simulink model "voll_bridge_tobias"  (R2026b)
settings: Solver=VariableStepAuto
undefined symbols (not defined in the file): C_in_filter, Delta, L, L1, L2, L_in_filter, Lm, N, n, N_points, R1, R2, R_in_filter, RFe, RLrp, TA
libraries: simulink x6, SDE_Blockset x1
settings Model: Creator=trainer  LastModifiedBy=d.bagnara
settings OptimizationCC: ReuseModelBlockBuffer=off

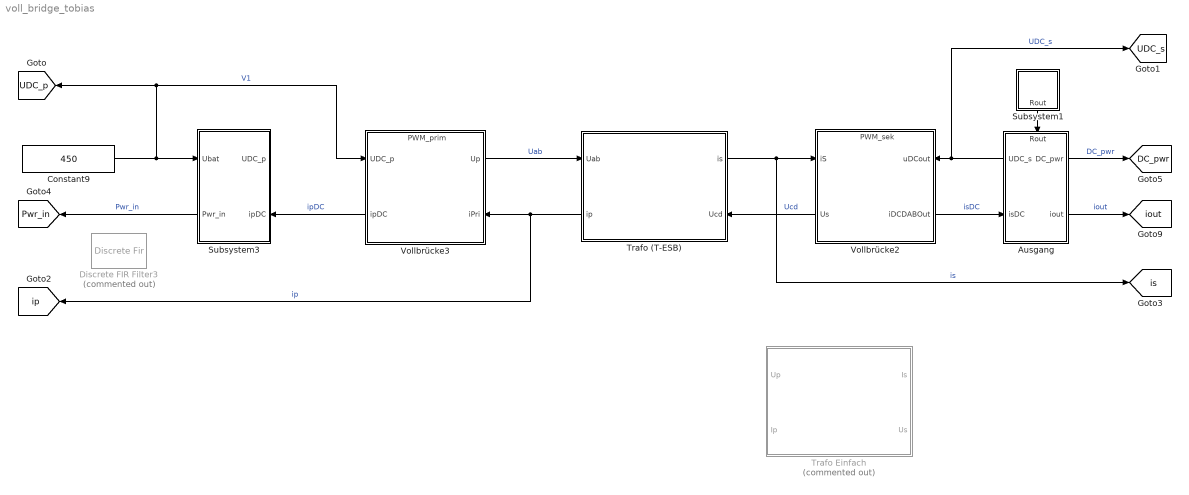
== system voll_bridge_tobias ==
  Ausgang : Subsystem
      settings: PortSchema="{\"entries\":[{\"content\":{\"sides\":[{\"content\":{\"connectorIds\":[\"Out3\",\"In1\"]},\"type\":\"ConnectorPlacement.EquallySpacedRectSide\",\"uuid\":\"3e2cff53-c875-49c6-8474-afa1ed1193a6\"},{\"content\":{\"connectorIds\":[\"Out1\",\"Out2\"],\"side\":\"RIGHT\"},\"type\":\"ConnectorPlacement.EquallySpacedRectSide\",\"uuid\":\"9e2ae12c-269a-4542-b310-d161ff5322e5\"},{\"content\":{\"connectorIds\":[\"In2\"],\"side\":\"TOP\"},\"type\":\"ConnectorPlacement.EquallySpacedRectSide\",\"uuid\":\"7466d0b4-47a5-439f-b3f3-5fed0d3de2ac\"}]},\"type\":\"ConnectorPlacement.EquallySpacedConnector\",\"uuid\":\"f94e0f93-850d-4090-9895-e2c6fde01ad6\"}],\"packageUris\":[\"http://schema.mathworks.com/mf0/Connector/R2020b\"],\"version\":\"1.0\"}"
  Constant9 : Constant  Value=450  OutDataTypeStr=S_F32
  Discrete FIR Filter3 : DiscreteFir  Commented=on  Coefficients=ones(1,N_points)/N_points  OutDataTypeStr=Inherit: Same as accumulator
  Subsystem1 : Subsystem
  Subsystem3 : Subsystem
      settings: PortSchema="{\"entries\":[{\"content\":{\"sides\":[{\"content\":{\"connectorIds\":[\"In1\",\"Out2\"]},\"type\":\"ConnectorPlacement.EquallySpacedRectSide\",\"uuid\":\"80c5ed0c-5841-4938-b898-84137f6d9c34\"},{\"content\":{\"connectorIds\":[\"Out1\",\"In2\"],\"side\":\"RIGHT\"},\"type\":\"ConnectorPlacement.EquallySpacedRectSide\",\"uuid\":\"8c17f11a-4998-4b66-b746-a293eee14202\"},{\"content\":{\"connectorIds\":[],\"side\":\"TOP\"},\"type\":\"ConnectorPlacement.EquallySpacedRectSide\",\"uuid\":\"e60db4c2-c92c-402f-8091-b49c7a789db5\"}]},\"type\":\"ConnectorPlacement.EquallySpacedConnector\",\"uuid\":\"558de1e2-c2ec-4343-96f3-e5efd467d9a7\"}],\"packageUris\":[\"http://schema.mathworks.com/mf0/Connector/R2020b\"],\"version\":\"1.0\"}"
  Trafo (T-ESB) : Subsystem
      settings: PortSchema="{\"entries\":[{\"content\":{\"sides\":[{\"content\":{\"connectorIds\":[\"In1\",\"Out2\"]},\"type\":\"ConnectorPlacement.EquallySpacedRectSide\",\"uuid\":\"6e81ceeb-0363-463f-984b-d2d8288a5ec4\"},{\"content\":{\"connectorIds\":[\"Out1\",\"In2\"],\"side\":\"RIGHT\"},\"type\":\"ConnectorPlacement.EquallySpacedRectSide\",\"uuid\":\"b30afd59-af09-43dc-9a37-2f5643c5d178\"},{\"content\":{\"connectorIds\":[],\"side\":\"TOP\"},\"type\":\"ConnectorPlacement.EquallySpacedRectSide\",\"uuid\":\"a71b4fb2-5a5a-43bb-9a64-a7dea3e55af5\"}]},\"type\":\"ConnectorPlacement.EquallySpacedConnector\",\"uuid\":\"85fc6124-daf2-4d92-a632-153b83626f2a\"}],\"packageUris\":[\"http://schema.mathworks.com/mf0/Connector/R2020b\"],\"version\":\"1.0\"}"
  Trafo Einfach : Subsystem  Commented=on
      settings: PortSchema="{\"entries\":[{\"content\":{\"sides\":[{\"content\":{\"connectorIds\":[\"In1\",\"Out2\"]},\"type\":\"ConnectorPlacement.EquallySpacedRectSide\",\"uuid\":\"c971f182-6d77-4937-8b05-b79f55e4c806\"},{\"content\":{\"connectorIds\":[\"Out1\",\"In2\"],\"side\":\"RIGHT\"},\"type\":\"ConnectorPlacement.EquallySpacedRectSide\",\"uuid\":\"37e64967-fcec-4802-beb3-69154f28263c\"},{\"content\":{\"connectorIds\":[],\"side\":\"TOP\"},\"type\":\"ConnectorPlacement.EquallySpacedRectSide\",\"uuid\":\"e411a49c-daa7-47d0-8386-3b1061192469\"},{\"content\":{\"connectorIds\":[],\"side\":\"BOTTOM\"},\"type\":\"ConnectorPlacement.EquallySpacedRectSide\",\"uuid\":\"ba50093e-ff36-4075-81bf-05719850c996\"}]},\"type\":\"ConnectorPlacement.EquallySpacedConnector\",\"uuid\":\"82c6f70e-365e-41e7-aef8-e59438ced761\"}],\"packageUris\":[\"http://schema.mathworks.com/mf0/Connector/R2020b\"],\"version\":\"1.0\"}"
  Vollbrücke2 : Subsystem
      settings: PortSchema="{\"entries\":[{\"content\":{\"sides\":[{\"content\":{\"connectorIds\":[\"In1\",\"Out2\"]},\"type\":\"ConnectorPlacement.EquallySpacedRectSide\",\"uuid\":\"b2581c16-97fc-43c2-9374-a6229b1b4c11\"},{\"content\":{\"connectorIds\":[\"In3\",\"Out1\"],\"side\":\"RIGHT\"},\"type\":\"ConnectorPlacement.EquallySpacedRectSide\",\"uuid\":\"06f310f8-024e-445b-b4e4-58d56c4e10df\"},{\"content\":{\"connectorIds\":[\"In2\"],\"side\":\"TOP\"},\"type\":\"ConnectorPlacement.EquallySpacedRectSide\",\"uuid\":\"c56b8861-8968-41d2-9579-8e1534e46433\"}]},\"type\":\"ConnectorPlacement.EquallySpacedConnector\",\"uuid\":\"550ed9c8-70a1-48c7-a2e5-e55cd52d4178\"}],\"packageUris\":[\"http://schema.mathworks.com/mf0/Connector/R2020b\"],\"version\":\"1.0\"}"
  Vollbrücke3 : Subsystem
      settings: PortSchema="{\"entries\":[{\"content\":{\"sides\":[{\"content\":{\"connectorIds\":[\"In1\",\"Out2\"]},\"type\":\"ConnectorPlacement.EquallySpacedRectSide\",\"uuid\":\"b2581c16-97fc-43c2-9374-a6229b1b4c11\"},{\"content\":{\"connectorIds\":[\"Out1\",\"In3\"],\"side\":\"RIGHT\"},\"type\":\"ConnectorPlacement.EquallySpacedRectSide\",\"uuid\":\"06f310f8-024e-445b-b4e4-58d56c4e10df\"},{\"content\":{\"connectorIds\":[\"In2\"],\"side\":\"TOP\"},\"type\":\"ConnectorPlacement.EquallySpacedRectSide\",\"uuid\":\"c56b8861-8968-41d2-9579-8e1534e46433\"}]},\"type\":\"ConnectorPlacement.EquallySpacedConnector\",\"uuid\":\"550ed9c8-70a1-48c7-a2e5-e55cd52d4178\"}],\"packageUris\":[\"http://schema.mathworks.com/mf0/Connector/R2020b\"],\"version\":\"1.0\"}"
  tag scope: DC_pwr=global, Pwr_in=global, UDC_p=global, UDC_s=global, iout=global, ip=global, is=global
  wires:
  Trafo (T-ESB)/1(is) -> [is], Vollbrücke2/1(iS)  "is"
  Trafo (T-ESB)/2(ip) -> [ip], Vollbrücke3/3(iPri)  "ip"
  Subsystem1/1(Rout) -> Ausgang/2(Rout)
  Vollbrücke3/1(Up) -> Trafo (T-ESB)/1(Uab)  "Uab"
  Ausgang/2(iout) -> [iout]  "iout"
  Vollbrücke2/2(Us) -> Trafo (T-ESB)/2(Ucd)  "Ucd"
  Vollbrücke2/1(iDCDABOut) -> Ausgang/1(isDC)  "isDC"
  Constant9/1 -> [UDC_p], Vollbrücke3/1(UDC_p), Subsystem3/1(Ubat)  "V1"
  Vollbrücke3/2(ipDC) -> Subsystem3/2(ipDC)  "ipDC"
  Ausgang/1(DC_pwr) -> [DC_pwr]  "DC_pwr"
  Ausgang/3(UDC_s) -> [UDC_s], Vollbrücke2/3(uDCout)  "UDC_s"
  Subsystem3/2(Pwr_in) -> [Pwr_in]  "Pwr_in"

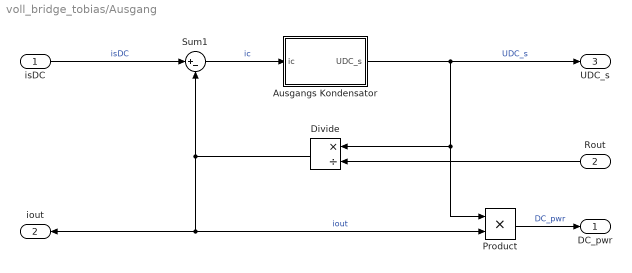
== system voll_bridge_tobias/Ausgang ==
  isDC : Inport
  Rout : Inport  Port=2
  Ausgangs Kondensator : Subsystem
  Divide : Product  Inputs=*/
  Product : Product
  Sum1 : Sum  Inputs=|+-
  DC_pwr : Outport
  iout : Outport  Port=2
  UDC_s : Outport  Port=3
  wires:
  Sum1/1 -> Ausgangs Kondensator/1(ic)  "ic"
  isDC/1 -> Sum1/1  "isDC"
  Divide/1 -> iout/1, Product/2, Sum1/2  "iout"
  Ausgangs Kondensator/1(UDC_s) -> UDC_s/1, Divide/1, Product/1  "UDC_s"
  Product/1 -> DC_pwr/1  "DC_pwr"
  Rout/1 -> Divide/2

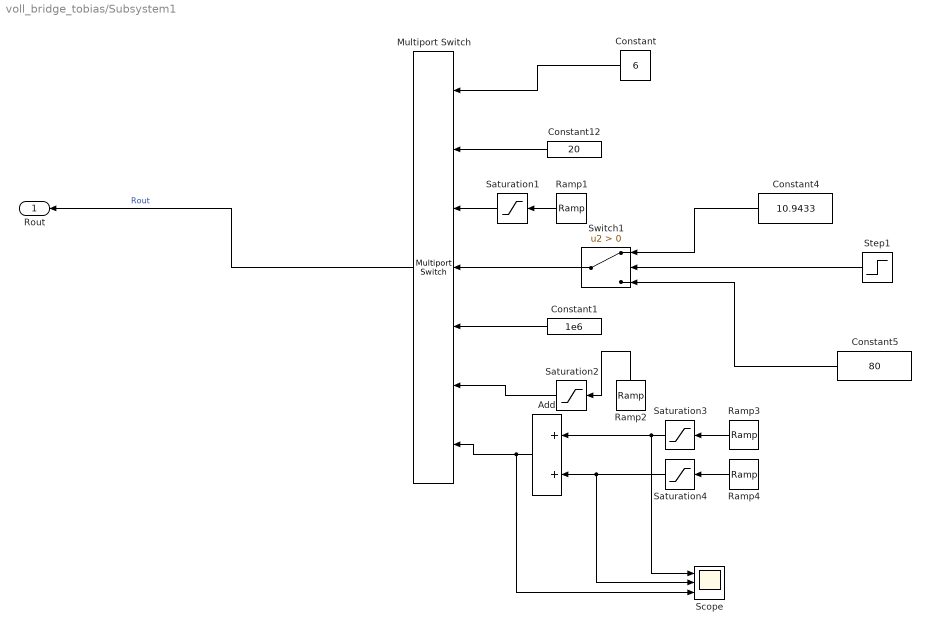
== system voll_bridge_tobias/Subsystem1 ==
  Add : Sum
  Constant : Constant  Value=6
  Constant1 : Constant  Value=1e6
  Constant12 : Constant  Value=20
  Constant4 : Constant  Value=10.9433
  Constant5 : Constant  Value=80
  Multiport Switch : SDE_Blockset/Signal Routing/Multiport Switch  DataPortOrder=One-based contiguous  Inputs=6  DataPortIndices={1,2,3}  DataPortForDefault=Last data port
      settings: SourceProductName=SDE_Blockset
  Ramp1 : simulink/Sources/Ramp  slope=-7450  start=0.005  InitialOutput=84.5
  Ramp2 : simulink/Sources/Ramp  slope=-1000  start=0.005  InitialOutput=20
  Ramp3 : simulink/Sources/Ramp  slope=-7450*2  start=0.005  InitialOutput=84.5
  Ramp4 : simulink/Sources/Ramp  slope=7450*2  start=0.02  InitialOutput=0
  Saturation1 : Saturate  UpperLimit=100  LowerLimit=10.9
  Saturation2 : Saturate  UpperLimit=100  LowerLimit=10.9
  Saturation3 : Saturate  UpperLimit=100  LowerLimit=10.9
  Saturation4 : Saturate  UpperLimit=84.5-10  LowerLimit=0
  Scope : Scope  NumInputPorts=3
      settings: ActiveDisplayYMinimum=1.7  ActiveDisplayYMaximum=93.7
  Step1 : Step  Time=0.005  SampleTime=0
  Switch1 : Switch  Criteria=u2 > Threshold  SaturateOnIntegerOverflow=off  InputSameDT=off
  Rout : Outport
  wires:
  Ramp1/1 -> Saturation1/1
  Constant4/1 -> Switch1/1
  Step1/1 -> Switch1/2
  Constant5/1 -> Switch1/3
  Constant12/1 -> Multiport Switch/2
  Saturation1/1 -> Multiport Switch/3
  Switch1/1 -> Multiport Switch/4
  Multiport Switch/1 -> Rout/1  "Rout"
  Constant/1 -> Multiport Switch/1
  Constant1/1 -> Multiport Switch/5
  Ramp2/1 -> Saturation2/1
  Saturation2/1 -> Multiport Switch/6
  Ramp3/1 -> Saturation3/1
  Add/1 -> Scope/3, Multiport Switch/7
  Saturation3/1 -> Scope/1, Add/1
  Saturation4/1 -> Scope/2, Add/2
  Ramp4/1 -> Saturation4/1

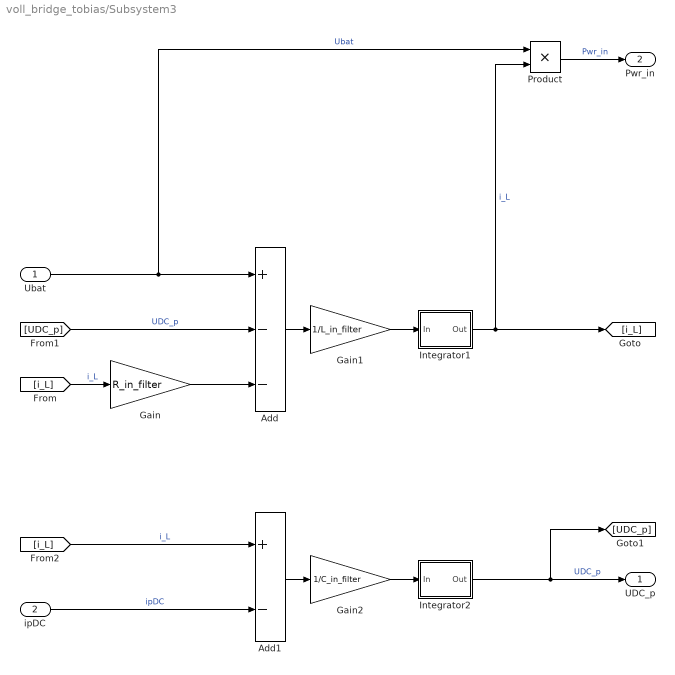
== system voll_bridge_tobias/Subsystem3 ==
  Ubat : Inport
  ipDC : Inport  Port=2
  Add : Sum  Inputs=+--
  Add1 : Sum  Inputs=+-
  Gain : Gain  Gain=R_in_filter
  Gain1 : Gain  Gain=1/L_in_filter
  Gain2 : Gain  Gain=1/C_in_filter
  Integrator1 : Subsystem
  Integrator2 : Subsystem
  Product : Product
  UDC_p : Outport
  Pwr_in : Outport  Port=2
  wires:
  Product/1 -> Pwr_in/1  "Pwr_in"
  ipDC/1 -> Add1/2  "ipDC"
  [i_L] -> Add1/1  "i_L"
  Gain2/1 -> Integrator2/1(In)
  Gain1/1 -> Integrator1/1(In)
  [UDC_p] -> Add/2  "UDC_p"
  [i_L] -> Gain/1  "i_L"
  Ubat/1 -> Add/1, Product/1  "Ubat"
  Add1/1 -> Gain2/1
  Integrator2/1(Out) -> UDC_p/1, [UDC_p]  "UDC_p"
  Integrator1/1(Out) -> [i_L], Product/2  "i_L"
  Add/1 -> Gain1/1
  Gain/1 -> Add/3

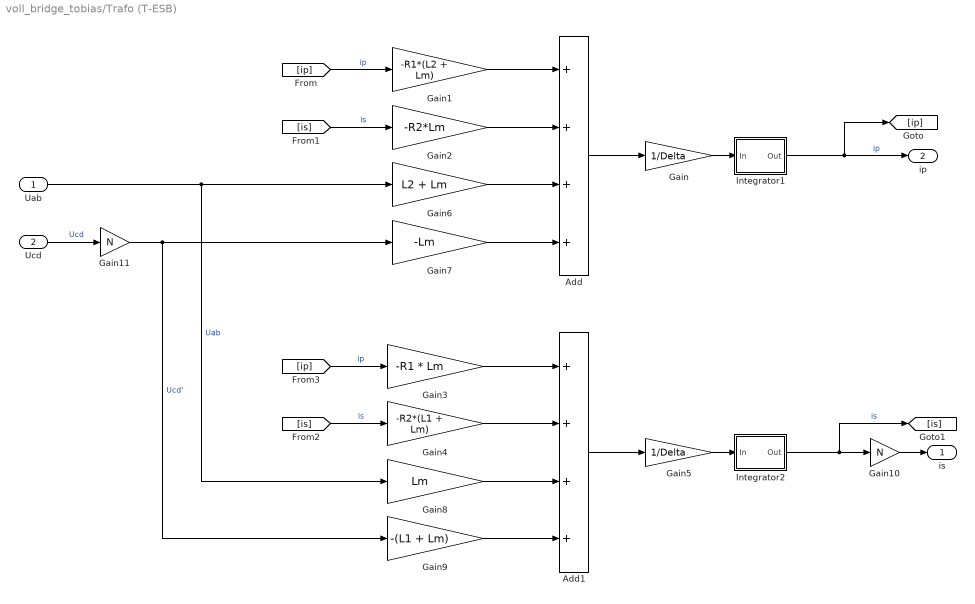
== system voll_bridge_tobias/Trafo (T-ESB) ==
  Uab : Inport
  Ucd : Inport  Port=2
  Add : Sum  Inputs=++++
  Add1 : Sum  Inputs=++++
  Gain : Gain  Gain=1/Delta
  Gain1 : Gain  Gain=-R1*(L2 + Lm)
  Gain10 : Gain  Gain=N
  Gain11 : Gain  Gain=N
  Gain2 : Gain  Gain=-R2*Lm
  Gain3 : Gain  Gain=-R1 * Lm
  Gain4 : Gain  Gain=-R2*(L1 + Lm)
  Gain5 : Gain  Gain=1/Delta
  Gain6 : Gain  Gain=L2 + Lm
  Gain7 : Gain  Gain=-Lm
  Gain8 : Gain  Gain=Lm
  Gain9 : Gain  Gain=-(L1 + Lm)
  Integrator1 : Subsystem
  Integrator2 : Subsystem
  is : Outport
  ip : Outport  Port=2
  wires:
  [ip] -> Gain1/1  "ip"
  Integrator2/1(Out) -> Gain10/1, [is]  "is"
  Gain2/1 -> Add/2
  Gain6/1 -> Add/3
  Gain4/1 -> Add1/2
  Gain9/1 -> Add1/4
  Gain/1 -> Integrator1/1(In)
  [is] -> Gain2/1  "is"
  [ip] -> Gain3/1  "ip"
  Gain1/1 -> Add/1
  Add/1 -> Gain/1
  [is] -> Gain4/1  "is"
  Add1/1 -> Gain5/1
  Gain8/1 -> Add1/3
  Gain7/1 -> Add/4
  Gain5/1 -> Integrator2/1(In)
  Ucd/1 -> Gain11/1  "Ucd"
  Gain3/1 -> Add1/1
  Integrator1/1(Out) -> ip/1, [ip]  "ip"
  Uab/1 -> Gain6/1, Gain8/1  "Uab"
  Gain10/1 -> is/1
  Gain11/1 -> Gain9/1, Gain7/1  "Ucd'"

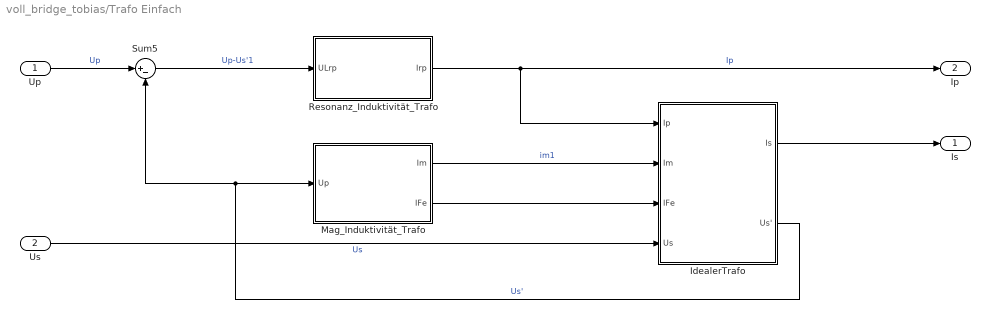
== system voll_bridge_tobias/Trafo Einfach ==
  Up : Inport
  Us : Inport  Port=2
  IdealerTrafo : Subsystem
  Mag_Induktivität_Trafo : Subsystem
  Resonanz_Induktivität_Trafo : Subsystem
  Sum5 : Sum  Inputs=|+-
  Is : Outport
  Ip : Outport  Port=2
  wires:
  Mag_Induktivität_Trafo/1(Im) -> IdealerTrafo/2(Im)  "im1"
  IdealerTrafo/2(Us') -> Sum5/2, Mag_Induktivität_Trafo/1(Up)  "Us'"
  Resonanz_Induktivität_Trafo/1(Irp) -> Ip/1, IdealerTrafo/1(Ip)  "Ip"
  Mag_Induktivität_Trafo/2(IFe) -> IdealerTrafo/3(IFe)
  Up/1 -> Sum5/1  "Up"
  Us/1 -> IdealerTrafo/4(Us)  "Us"
  IdealerTrafo/1(Is) -> Is/1
  Sum5/1 -> Resonanz_Induktivität_Trafo/1(ULrp)  "Up-Us'1"

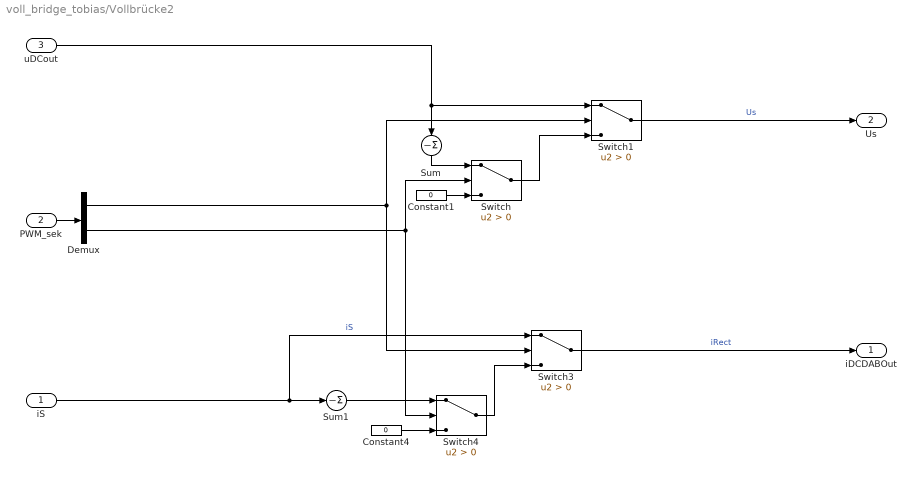
== system voll_bridge_tobias/Vollbrücke2 ==
  iS : Inport
  PWM_sek : Inport  Port=2
  uDCout : Inport  Port=3
  Constant1 : Constant  Value=0
  Constant4 : Constant  Value=0
  Demux : Demux  Outputs=2
  Sum : Sum  Inputs=-
  Sum1 : Sum  Inputs=-
  Switch{,1,3..4} (4 alike) : Switch  Criteria=u2 > Threshold  SaturateOnIntegerOverflow=off  InputSameDT=off
  iDCDABOut : Outport  VectorParamsAs1DForOutWhenUnconnected=off
  Us : Outport  Port=2  VectorParamsAs1DForOutWhenUnconnected=off
  wires:
  Switch4/1 -> Switch3/3
  Constant4/1 -> Switch4/3
  Switch/1 -> Switch1/3
  iS/1 -> Switch3/1, Sum1/1  "iS"
  Constant1/1 -> Switch/3
  Sum1/1 -> Switch4/1
  Sum/1 -> Switch/1
  uDCout/1 -> Switch1/1, Sum/1
  PWM_sek/1 -> Demux/1
  Demux/1 -> Switch1/2, Switch3/2
  Demux/2 -> Switch4/2, Switch/2
  Switch1/1 -> Us/1  "Us"
  Switch3/1 -> iDCDABOut/1  "iRect"

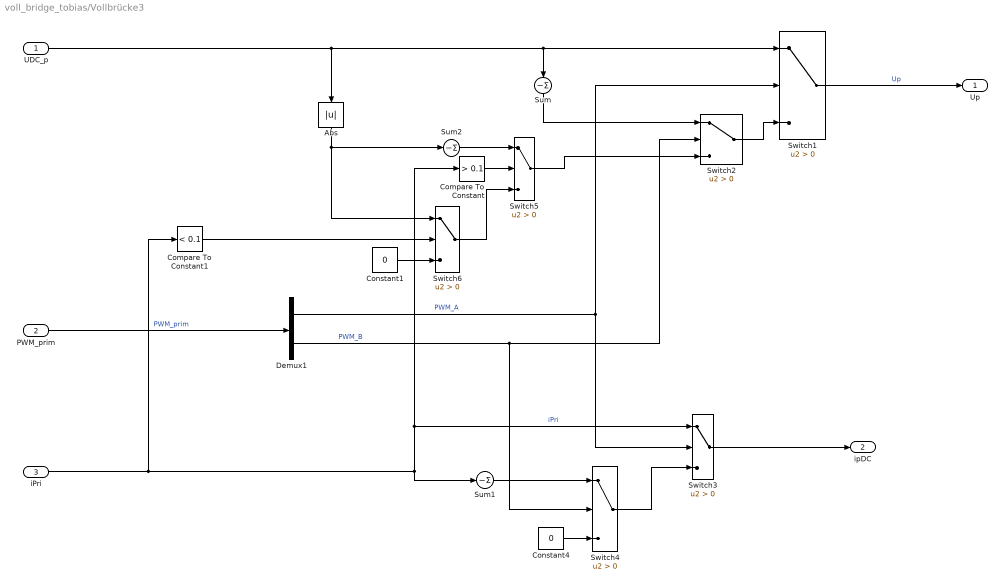
== system voll_bridge_tobias/Vollbrücke3 ==
  UDC_p : Inport
  PWM_prim : Inport  Port=2
  iPri : Inport  Port=3
  Abs : Abs  SaturateOnIntegerOverflow=off
  Compare To Constant : simulink/Logic and Bit Operations/Compare To Constant  relop=>  const=0.1  OutDataTypeStr=boolean
  Compare To Constant1 : simulink/Logic and Bit Operations/Compare To Constant  relop=<  const=0.1  OutDataTypeStr=boolean
  Constant1 : Constant  Value=0
  Constant4 : Constant  Value=0
  Demux1 : Demux  Outputs=2
  Sum : Sum  Inputs=-
  Sum1 : Sum  Inputs=-
  Sum2 : Sum  Inputs=-
  Switch{1..6} (6 alike) : Switch  Criteria=u2 > Threshold  SaturateOnIntegerOverflow=off  InputSameDT=off
  Up : Outport  VectorParamsAs1DForOutWhenUnconnected=off
  ipDC : Outport  Port=2  VectorParamsAs1DForOutWhenUnconnected=off
  wires:
  Switch4/1 -> Switch3/3
  Constant4/1 -> Switch4/3
  Switch2/1 -> Switch1/3
  iPri/1 -> Sum1/1, Compare To Constant/1, Switch3/1, Compare To Constant1/1  "iPri"
  Switch5/1 -> Switch2/3
  Sum1/1 -> Switch4/1
  Sum/1 -> Switch2/1
  UDC_p/1 -> Switch1/1, Sum/1, Abs/1
  Demux1/1 -> Switch3/2, Switch1/2  "PWM_A"
  Demux1/2 -> Switch2/2, Switch4/2  "PWM_B"
  PWM_prim/1 -> Demux1/1  "PWM_prim"
  Compare To Constant/1 -> Switch5/2
  Switch6/1 -> Switch5/3
  Compare To Constant1/1 -> Switch6/2
  Constant1/1 -> Switch6/3
  Sum2/1 -> Switch5/1
  Abs/1 -> Sum2/1, Switch6/1
  Switch1/1 -> Up/1  "Up"
  Switch3/1 -> ipDC/1

== system voll_bridge_tobias/Ausgang/Ausgangs Kondensator ==
  ic : Inport
  Gain2 : Gain  Gain=1/33.6e-6
  Integrator : Subsystem
  UDC_s : Outport  VectorParamsAs1DForOutWhenUnconnected=off
  wires:
  ic/1 -> Gain2/1  "ic"
  Gain2/1 -> Integrator/1(In)
  Integrator/1(Out) -> UDC_s/1  "UDC_s"

== system voll_bridge_tobias/Subsystem3/Integrator1 ==
  In : Inport
  Gain1 : Gain  Gain=TA
  Sum4 : Sum  Inputs=|++
  Unit Delay : UnitDelay  InitialCondition=450  SampleTime=-1
      settings: AttributesFormatString=%<InitialCondition>
  Out : Outport
  wires:
  In/1 -> Gain1/1
  Unit Delay/1 -> Out/1, Sum4/2
  Sum4/1 -> Unit Delay/1
  Gain1/1 -> Sum4/1

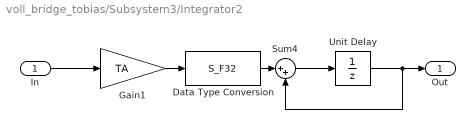
== system voll_bridge_tobias/Subsystem3/Integrator2 ==
  In : Inport
  Data Type Conversion : DataTypeConversion  OutDataTypeStr=S_F32  SaturateOnIntegerOverflow=off  RndMeth=Floor
  Gain1 : Gain  Gain=TA
  Sum4 : Sum  Inputs=|++
  Unit Delay : UnitDelay  InitialCondition=450  SampleTime=-1
      settings: AttributesFormatString=%<InitialCondition>
  Out : Outport
  wires:
  Data Type Conversion/1 -> Sum4/1
  Gain1/1 -> Data Type Conversion/1
  Sum4/1 -> Unit Delay/1
  Unit Delay/1 -> Sum4/2, Out/1
  In/1 -> Gain1/1

== system voll_bridge_tobias/Trafo (T-ESB)/Integrator1 ==
  In : Inport
  Gain1 : Gain  Gain=TA
  Sum4 : Sum  Inputs=|++
  Unit Delay : UnitDelay  SampleTime=-1
      settings: AttributesFormatString=%<InitialCondition>
  Out : Outport
  wires:
  Gain1/1 -> Sum4/1
  Sum4/1 -> Unit Delay/1
  Unit Delay/1 -> Sum4/2, Out/1
  In/1 -> Gain1/1

== system voll_bridge_tobias/Trafo (T-ESB)/Integrator2 ==
  In : Inport
  Gain1 : Gain  Gain=TA
  Sum4 : Sum  Inputs=|++
  Unit Delay : UnitDelay  SampleTime=-1
      settings: AttributesFormatString=%<InitialCondition>
  Out : Outport
  wires:
  In/1 -> Gain1/1
  Unit Delay/1 -> Out/1, Sum4/2
  Sum4/1 -> Unit Delay/1
  Gain1/1 -> Sum4/1

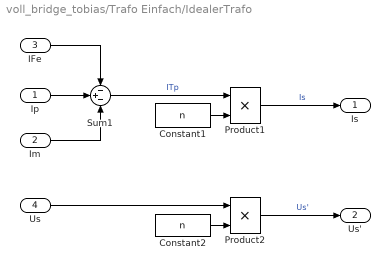
== system voll_bridge_tobias/Trafo Einfach/IdealerTrafo ==
  Ip : Inport
  Im : Inport  Port=2
  IFe : Inport  Port=3
  Us : Inport  Port=4
  Constant1 : Constant  InitFcn=%set_param(gcb, 'AttributesFormatString',['= ' num2str(eval(get_param(gcb,'Value')))])  Value=n
      settings: AttributesFormatString== 0.99499
  Constant2 : Constant  InitFcn=%set_param(gcb, 'AttributesFormatString',['= ' num2str(eval(get_param(gcb,'Value')))])  Value=n
      settings: AttributesFormatString== 0.99499
  Product1 : Product  Inputs=**
  Product2 : Product  Inputs=**
  Sum1 : Sum  Inputs=-+-
  Is : Outport  VectorParamsAs1DForOutWhenUnconnected=off
  Us' : Outport  Port=2  VectorParamsAs1DForOutWhenUnconnected=off
  wires:
  Constant2/1 -> Product2/2
  Constant1/1 -> Product1/2
  Im/1 -> Sum1/3
  Sum1/1 -> Product1/1  "ITp"
  Ip/1 -> Sum1/2
  Product2/1 -> Us'/1  "Us'"
  Us/1 -> Product2/1
  IFe/1 -> Sum1/1
  Product1/1 -> Is/1  "Is"

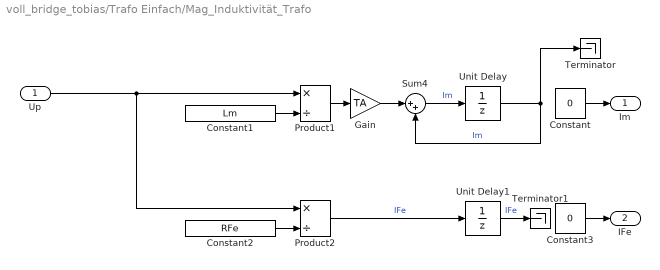
== system voll_bridge_tobias/Trafo Einfach/Mag_Induktivität_Trafo ==
  Up : Inport
  Constant : Constant  Value=0
  Constant1 : Constant  InitFcn=%set_param(gcb, 'AttributesFormatString',['= ' num2str(eval(get_param(gcb,'Value')))])  Value=Lm
      settings: AttributesFormatString== 0.0005
  Constant2 : Constant  InitFcn=set_param(gcb, 'AttributesFormatString',['= ' num2str(eval(get_param(gcb,'Value')))])  Value=RFe
      settings: AttributesFormatString== 1000000
  Constant3 : Constant  Value=0
  Gain : Gain  Gain=TA
  Product1 : Product  Inputs=*/
  Product2 : Product  Inputs=*/
  Sum4 : Sum  Inputs=|++
  Terminator : Terminator
  Terminator1 : Terminator
  Unit Delay : UnitDelay  SampleTime=-1
      settings: AttributesFormatString=%<X0>
  Unit Delay1 : UnitDelay  SampleTime=-1
      settings: AttributesFormatString=%<X0>
  Im : Outport  VectorParamsAs1DForOutWhenUnconnected=off
  IFe : Outport  Port=2  VectorParamsAs1DForOutWhenUnconnected=off
  wires:
  Constant2/1 -> Product2/2
  Product1/1 -> Gain/1
  Constant1/1 -> Product1/2
  Sum4/1 -> Unit Delay/1  "Im"
  Up/1 -> Product1/1, Product2/1
  Unit Delay/1 -> Terminator/1, Sum4/2  "Im"
  Gain/1 -> Sum4/1
  Product2/1 -> Unit Delay1/1  "IFe"
  Unit Delay1/1 -> Terminator1/1  "IFe"
  Constant/1 -> Im/1
  Constant3/1 -> IFe/1

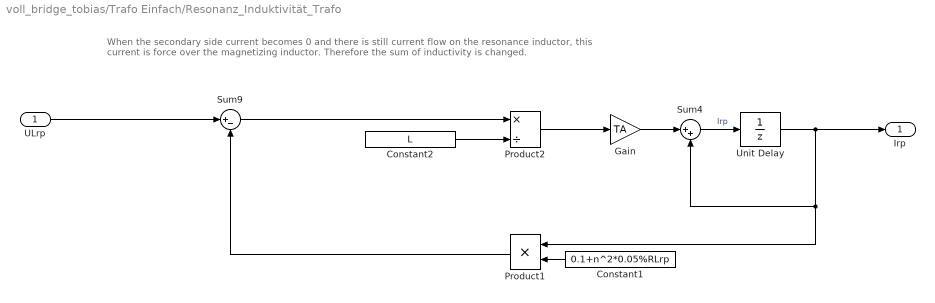
== system voll_bridge_tobias/Trafo Einfach/Resonanz_Induktivität_Trafo ==
  note: When the secondary side current becomes 0 and there is still current flow on the resonance inductor, this current is force over the magnetizing inductor.
      | Therefore the sum of inductivity is changed.
  ULrp : Inport
  Constant1 : Constant  InitFcn=set_param(gcb, 'AttributesFormatString',['= ' num2str(eval(get_param(gcb,'Value')))])  Value=0.1+n^2*0.05%RLrp
      settings: AttributesFormatString== 0.15
  Constant2 : Constant  InitFcn=%set_param(gcb, 'AttributesFormatString',['= ' num2str(eval(get_param(gcb,'Value')))])  Value=L
  Gain : Gain  Gain=TA
  Product1 : Product  Inputs=**
  Product2 : Product  Inputs=*/
  Sum4 : Sum  Inputs=|++
  Sum9 : Sum  Inputs=|+-
  Unit Delay : UnitDelay  SampleTime=-1
      settings: AttributesFormatString=%<X0>
  Irp : Outport  VectorParamsAs1DForOutWhenUnconnected=off
  wires:
  Constant2/1 -> Product2/2
  Constant1/1 -> Product1/2
  Gain/1 -> Sum4/1
  ULrp/1 -> Sum9/1
  Sum4/1 -> Unit Delay/1  "Irp"
  Sum9/1 -> Product2/1
  Product2/1 -> Gain/1
  Unit Delay/1 -> Irp/1, Sum4/2, Product1/1
  Product1/1 -> Sum9/2

== system voll_bridge_tobias/Ausgang/Ausgangs Kondensator/Integrator ==
  In : Inport
  Gain1 : Gain  Gain=TA
  Sum4 : Sum  Inputs=|++
  Unit Delay : UnitDelay  InitialCondition=400  SampleTime=-1
      settings: AttributesFormatString=%<InitialCondition>
  Out : Outport
  wires:
  Gain1/1 -> Sum4/1
  Sum4/1 -> Unit Delay/1
  Unit Delay/1 -> Sum4/2, Out/1
  In/1 -> Gain1/1
